simulink model "VTS_challenge_2021"  (R2019b)
settings: Solver=ode1  StartTime=0.0  StopTime=SIMULPARAM.T_end  FixedStep=SIMULPARAM.Ts  RelTol=1e-3
undefined symbols (not defined in the file or in its folder): BAT, CHAp, EM1, EM2, EMS, MTp, RDp, Speed_control, SPEEDCONTROL
libraries: simulink x3
(part 1 of 2)
settings Model: Creator=baohu  LastModifiedBy=HIEU
settings DataIOCC: ReturnWorkspaceOutputs=off
settings OptimizationCC: LifeSpan=inf
settings DebuggingCC: SFExecutionAtInitializationDiag=none  ArithmeticOperatorsInVariantConditions=warning
settings HardwareCC: ProdBitPerSizeT=32  ProdBitPerPtrDiffT=32  ProdWordSize=32  ProdHWDeviceType=Specified
settings ModelReferenceCC: EnableRefExpFcnMdlSchedulingChecks=off
settings SFSimCC: SimUseLocalCustomCode=off  CustomCodeUndefinedFunction=UseInterfaceOnly
settings RTWCC: RTWUseLocalCustomCode=off
settings CodeAppCC: StateflowObjectComments=on

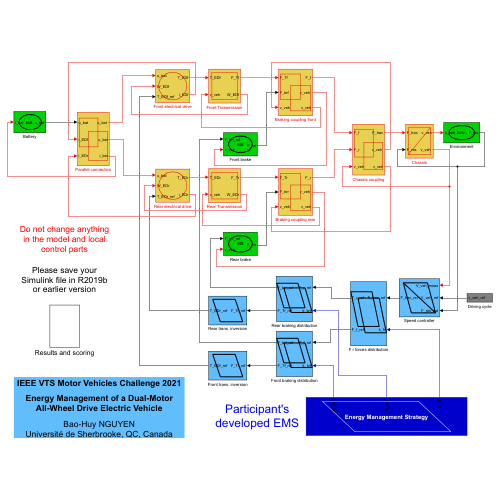
[thumbnail: Simulink's stored preview of the top-level diagram]
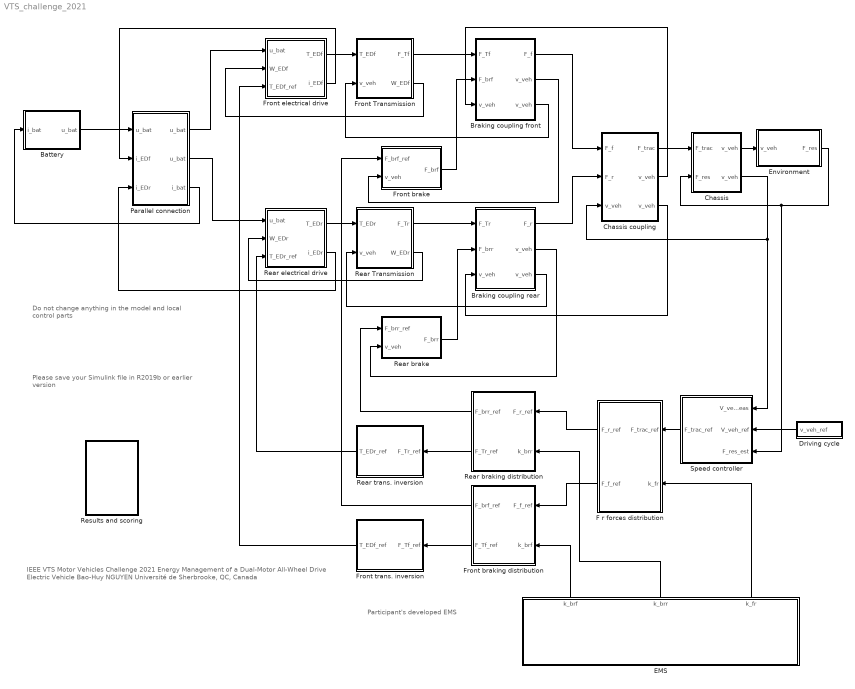
== system VTS_challenge_2021 ==
  note: Do not change anything in the model and local control parts
  note: Participant's developed EMS
  note: IEEE VTS Motor Vehicles Challenge 2021
      |
      | Energy Management of a Dual-Motor
      | All-Wheel Drive Electric Vehicle
      |
      | Bao-Huy NGUYEN
      | Université de Sherbrooke, QC, Canada
  note: Please save your Simulink file in R2019b or earlier version
  Battery : Subsystem
      mask Display:
      | plot(0,0,100,100, 1.2*[50,57.68,60.77,63.08,64.97,66.58,68,69.26,70.4, 	71.42,72.36,78.28,80,78.28,72.36,71.42,70.4, 	69.26,68,66.58,64.97,63.08,60.77,57.68,50,42.32, 	39.23,36.92,35.03,33.42,32,30.74,29.6,28.58, 	27.64,21.72,20,21.72,27.64,28.58,29.6,30.74,32, 	33.42,35.03,36.92,39.23,42.32,50]-10, 1.2*[20,21,22,23,24,25,26,27,28,29,30,40,50,60,70,71,72, 	73,74,75,76,77,78,79,80,79,78,77,76,75,74,73,72, 	71,70,60,50,40,30,29,28,27,26,25,24,23,22,21,20]-10)
      | disp('Bat.')
  Braking coupling front : Subsystem  mask(CM){}
      mask Display: plot(0,0,100,100,[35,35,95,95,35],[65,10,10,65,65], [5,5,65,65,5],[90,35,35,90,90])
  Braking coupling rear : Subsystem  mask(CM){}
      mask Display: plot(0,0,100,100,[35,35,95,95,35],[65,10,10,65,65], [5,5,65,65,5],[90,35,35,90,90])
  Chassis : Subsystem  mask(CM){}
      mask Display: plot(0,0,100,100,[10,10,90,90,10],[90,10,10,90,90], [10,90],[10,90])
  Chassis coupling : Subsystem  mask(CM){}
      mask Display: plot(0,0,100,100,[35,35,95,95,35],[65,10,10,65,65], [5,5,65,65,5],[90,35,35,90,90])
  Driving cycle : Subsystem
  EMS : Subsystem
      mask Display:
      | color('white');
      | plot(0,0,100,100,[10,30,90,70,10],[90,10,10,90,90])
      | disp('Energy Management Strategy')
  Environment : Subsystem
      mask Display:
      | plot(0,0,100,100, 1.2*[50,57.68,60.77,63.08,64.97,66.58,68,69.26,70.4, 	71.42,72.36,78.28,80,78.28,72.36,71.42,70.4, 	69.26,68,66.58,64.97,63.08,60.77,57.68,50,42.32, 	39.23,36.92,35.03,33.42,32,30.74,29.6,28.58, 	27.64,21.72,20,21.72,27.64,28.58,29.6,30.74,32, 	33.42,35.03,36.92,39.23,42.32,50]-10, 1.2*[20,21,22,23,24,25,26,27,28,29,30,40,50,60,70,71,72, 	73,74,75,76,77,78,79,80,79,78,77,76,75,74,73,72, 	71,70,60,50,40,30,29,28,27,26,25,24,23,22,21,20]-10)
      | disp('Env.')
  F r forces distribution : Subsystem
      mask Display: plot(0,0,100,100,[20,40,100,80,20],[75,20,20,75,75], [0,20,80,60,0],[85,30,30,85,85])
  Front Transmission : Subsystem
      mask Display: plot(0,0,100,100,[10,10,90,90,10],[90,10,10,90,90])
  Front brake : Subsystem
      mask Display:
      | plot(0,0,100,100, 1.2*[50,57.68,60.77,63.08,64.97,66.58,68,69.26,70.4, 	71.42,72.36,78.28,80,78.28,72.36,71.42,70.4, 	69.26,68,66.58,64.97,63.08,60.77,57.68,50,42.32, 	39.23,36.92,35.03,33.42,32,30.74,29.6,28.58, 	27.64,21.72,20,21.72,27.64,28.58,29.6,30.74,32, 	33.42,35.03,36.92,39.23,42.32,50]-10, 1.2*[20,21,22,23,24,25,26,27,28,29,30,40,50,60,70,71,72, 	73,74,75,76,77,78,79,80,79,78,77,76,75,74,73,72, 	71,70,60,50,40,30,29,28,27,26,25,24,23,22,21,20]-10)
      | disp('MS')
  Front braking distribution : Subsystem
      mask Display: plot(0,0,100,100,[20,40,100,80,20],[75,20,20,75,75], [0,20,80,60,0],[85,30,30,85,85])
  Front electrical drive : Subsystem
      mask Display: plot(0,0,100,100, 1.4*[50,57.68,60.77,63.08,64.97,66.58,68,69.26,70.4, 	71.42,72.36,78.28,80,78.28,72.36,71.42,70.4, 	69.26,68,66.58,64.97,63.08,60.77,57.68,50,42.32, 	39.23,36.92,35.03,33.42,32,30.74,29.6,28.58, 	27.64,21.72,20,21.72,27.64,28.58,29.6,30.74,32, 	33.42,35.03,36.92,39.23,42.32,50]-20, 1.4*[20,21,22,23,24,25,26,27,28,29,30,40,50,60,70,71,72, 	73,74,75,76,77,78,79,80,79,78,77,76,75,74,73,72, 	71,70,60,50,40,30,29,28,27,26,25,24,23,22,21,20]-20)
  Front trans. inversion : Subsystem
      mask Display: plot(0,0,100,100,[10,30,90,70,10],[90,10,10,90,90])
  Parallel connection : Subsystem  mask(CM){}
      mask Display: plot(0,0,100,100,[35,35,95,95,35],[65,10,10,65,65], [5,5,65,65,5],[90,35,35,90,90])
  Rear Transmission : Subsystem
      mask Display: plot(0,0,100,100,[10,10,90,90,10],[90,10,10,90,90])
  Rear brake : Subsystem
      mask Display:
      | plot(0,0,100,100, 1.2*[50,57.68,60.77,63.08,64.97,66.58,68,69.26,70.4, 	71.42,72.36,78.28,80,78.28,72.36,71.42,70.4, 	69.26,68,66.58,64.97,63.08,60.77,57.68,50,42.32, 	39.23,36.92,35.03,33.42,32,30.74,29.6,28.58, 	27.64,21.72,20,21.72,27.64,28.58,29.6,30.74,32, 	33.42,35.03,36.92,39.23,42.32,50]-10, 1.2*[20,21,22,23,24,25,26,27,28,29,30,40,50,60,70,71,72, 	73,74,75,76,77,78,79,80,79,78,77,76,75,74,73,72, 	71,70,60,50,40,30,29,28,27,26,25,24,23,22,21,20]-10)
      | disp('MS')
  Rear braking distribution : Subsystem
      mask Display: plot(0,0,100,100,[20,40,100,80,20],[75,20,20,75,75], [0,20,80,60,0],[85,30,30,85,85])
  Rear electrical drive : Subsystem
      mask Display: plot(0,0,100,100, 1.4*[50,57.68,60.77,63.08,64.97,66.58,68,69.26,70.4, 	71.42,72.36,78.28,80,78.28,72.36,71.42,70.4, 	69.26,68,66.58,64.97,63.08,60.77,57.68,50,42.32, 	39.23,36.92,35.03,33.42,32,30.74,29.6,28.58, 	27.64,21.72,20,21.72,27.64,28.58,29.6,30.74,32, 	33.42,35.03,36.92,39.23,42.32,50]-20, 1.4*[20,21,22,23,24,25,26,27,28,29,30,40,50,60,70,71,72, 	73,74,75,76,77,78,79,80,79,78,77,76,75,74,73,72, 	71,70,60,50,40,30,29,28,27,26,25,24,23,22,21,20]-20)
  Rear trans. inversion : Subsystem
      mask Display: plot(0,0,100,100,[10,30,90,70,10],[90,10,10,90,90])
  Results and scoring : Subsystem
  Speed controller : Subsystem
      mask Display: plot(0,0,100,100, [10,30,90,70,10,90],[90,10,10,90,90,10])
  wires:
  Environment/1(F_res) -> Chassis/2(F_res), Speed controller/3(F_res_est)
  Chassis/1(v_veh) -> Environment/1(v_veh)
  Speed controller/1(F_trac_ref) -> F r forces distribution/1(F_trac_ref)
  Chassis/2("v_veh ") -> Chassis coupling/3(v_veh), Speed controller/1(V_veh_meas)
  Front Transmission/2(W_EDf) -> Front electrical drive/2(W_EDf)
  Battery/1(u_bat) -> Parallel connection/1(u_bat)
  Parallel connection/3(i_bat) -> Battery/1(i_bat)
  Rear electrical drive/2(i_EDr) -> Parallel connection/3(i_EDr)
  Front electrical drive/2(i_EDf) -> Parallel connection/2("i_EDf  ")
  Parallel connection/1("u_bat ") -> Front electrical drive/1(u_bat)
  Parallel connection/2(" u_bat") -> Rear electrical drive/1(u_bat)
  Front electrical drive/1(T_EDf) -> Front Transmission/1(T_EDf)
  Rear electrical drive/1(T_EDr) -> Rear Transmission/1(T_EDr)
  Rear Transmission/2(W_EDr) -> Rear electrical drive/2(W_EDr)
  Front Transmission/1(F_Tf) -> Braking coupling front/1(F_Tf)
  Front brake/1(F_brf) -> Braking coupling front/2(F_brf)
  Braking coupling front/3(" v_veh") -> Front Transmission/2(v_veh)
  Rear Transmission/1(F_Tr) -> Braking coupling rear/1(F_Tr)
  Rear brake/1(F_brr) -> Braking coupling rear/2(F_brr)
  Braking coupling rear/3(" v_veh") -> Rear Transmission/2(v_veh)
  Braking coupling rear/2("v_veh ") -> Rear brake/2(v_veh)
  Braking coupling front/2("v_veh ") -> Front brake/2(v_veh)
  Braking coupling front/1(F_f) -> Chassis coupling/1(F_f)
  Braking coupling rear/1(F_r) -> Chassis coupling/2(F_r)
  Chassis coupling/1(F_trac) -> Chassis/1(F_trac)
  Chassis coupling/2("v_veh ") -> Braking coupling front/3(v_veh)
  Chassis coupling/3(" v_veh") -> Braking coupling rear/3(v_veh)
  Front braking distribution/2(F_Tf_ref) -> Front trans. inversion/1(F_Tf_ref)
  Rear braking distribution/2(F_Tr_ref) -> Rear trans. inversion/1(F_Tr_ref)
  Rear trans. inversion/1(T_EDr_ref) -> Rear electrical drive/3(T_EDr_ref)
  Front trans. inversion/1(T_EDf_ref) -> Front electrical drive/3(T_EDf_ref)
  F r forces distribution/1(F_r_ref) -> Rear braking distribution/1(F_r_ref)
  F r forces distribution/2(F_f_ref) -> Front braking distribution/1(F_f_ref)
  Rear braking distribution/1(F_brr_ref) -> Rear brake/1(F_brr_ref)
  Front braking distribution/1(F_brf_ref) -> Front brake/1(F_brf_ref)
  EMS/3(k_fr) -> F r forces distribution/2(k_fr)
  EMS/2(k_brr) -> Rear braking distribution/2(k_brr)
  EMS/1(k_brf) -> Front braking distribution/2(k_brf)
  Driving cycle/1(v_veh_ref) -> Speed controller/2(V_veh_ref)

== system VTS_challenge_2021/Battery ==
  i_bat : Inport
  Air : Subsystem
      mask Display: plot(0,0,100,100, 1.2*[50,57.68,60.77,63.08,64.97,66.58,68,69.26,70.4, 	71.42,72.36,78.28,80,78.28,72.36,71.42,70.4, 	69.26,68,66.58,64.97,63.08,60.77,57.68,50,42.32, 	39.23,36.92,35.03,33.42,32,30.74,29.6,28.58, 	27.64,21.72,20,21.72,27.64,28.58,29.6,30.74,32, 	33.42,35.03,36.92,39.23,42.32,50]-10, 1.2*[20,21,22,23,24,25,26,27,28,29,30,40,50,60,70,71,72, 	73,74,75,76,77,78,79,80,79,78,77,76,75,74,73,72, 	71,70,60,50,40,30,29,28,27,26,25,24,23,22,21,20]-10)
  Cell ESR : Subsystem  mask(CM){}
      mask Display: plot(0,0,100,100, [50,57.68,60.77,63.08,64.97,66.58,68,69.26,70.4, 	71.42,72.36,78.28,80,78.28,72.36,71.42,70.4, 	69.26,68,66.58,64.97,63.08,60.77,57.68,50,42.32, 	39.23,36.92,35.03,33.42,32,30.74,29.6,28.58, 	27.64,21.72,20,21.72,27.64,28.58,29.6,30.74,32, 	33.42,35.03,36.92,39.23,42.32,50], [20,21,22,23,24,25,26,27,28,29,30,40,50,60,70,71,72, 	73,74,75,76,77,78,79,80,79,78,77,76,75,74,73,72, 	71,70,60,50,40,30,29,28,27,26,25,24,23,22,21,20]-15,  [50,57.68,60.77,63.08,64.97,66.58,68,69.26,70.4, 	71.42,72.36,78.28,80,78.28,72.36,71.42,70.4, 	69.26,68,66.58,64.97,63.08,60.77,57.68,50,42.32, 	39.23,36.92,35.03,33.42,32,30.74,29.6,28.58, 	27.64,21.72,20,21.72,27.64,28.58,29.6,30.74,32, 	33.42,35.03,36.92,39.23,42.32,50], [20,21,22,23,24,25,26,27,28,29,30,40,50,60,70,71,72, 	73,74,75,76,77,78,79,80,79,78,77,76,75,74,73,72, 	71,70,60,50,40,30,29,28,27,26,25,24,23,22,21,20]+15)
  Cell OCV : Subsystem
      mask Display: plot(0,0,100,100, 1.2*[50,57.68,60.77,63.08,64.97,66.58,68,69.26,70.4, 	71.42,72.36,78.28,80,78.28,72.36,71.42,70.4, 	69.26,68,66.58,64.97,63.08,60.77,57.68,50,42.32, 	39.23,36.92,35.03,33.42,32,30.74,29.6,28.58, 	27.64,21.72,20,21.72,27.64,28.58,29.6,30.74,32, 	33.42,35.03,36.92,39.23,42.32,50]-10, 1.2*[20,21,22,23,24,25,26,27,28,29,30,40,50,60,70,71,72, 	73,74,75,76,77,78,79,80,79,78,77,76,75,74,73,72, 	71,70,60,50,40,30,29,28,27,26,25,24,23,22,21,20]-10)
  Series parallel connection : Subsystem  mask(CM){}
      mask Display: plot(0,0,100,100, [10,10,90,90,10],[90,10,10,90,90], [10,90,10],[10,45,90])
  Thermal capacitance : Subsystem  mask(CM){}
      mask Display: plot(0,0,100,100,[10,10,90,90,10],[90,10,10,90,90], [10,90],[10,90])
  Thermal resistance : Subsystem
      mask Display: plot(0,0,100,100,[10,10,90,90,10],[90,10,10,90,90])
  u_bat : Outport  InitialOutput=0
  tag scope: i_bat=global, u_bat=global
  wires:
  i_bat/1 -> Series parallel connection/2(i_bat), [i_bat]
  Series parallel connection/1(u_bat) -> u_bat/1, [u_bat]
  Cell ESR/1(u_cell) -> Series parallel connection/1(u_cell)
  Series parallel connection/2("i_cell ") -> Cell ESR/3("i_cell ")
  Cell OCV/1(u_cell_OC) -> Cell ESR/1(u_cell_OC)
  Cell ESR/3(i_cell) -> Cell OCV/1(i_cell)
  Thermal resistance/1(q_sa) -> Air/1(q_sa)
  Air/1(T_air) -> Thermal resistance/2(T_air)
  Thermal resistance/2(q_cs) -> Thermal capacitance/2(q_cs)
  Thermal capacitance/1(T_cell) -> Thermal resistance/1(T_cell)
  Thermal capacitance/2(" T_cell ") -> Cell ESR/2(T_cell)
  Cell ESR/2(q_cell) -> Thermal capacitance/1(q_cell)

== system VTS_challenge_2021/Braking coupling front ==
  F_Tf : Inport
  F_brf : Inport  Port=2
  v_veh : Inport  Port=3
  Sum : Sum  Inputs=|++
  F_f : Outport  InitialOutput=0
  "v_veh " : Outport  Port=2  InitialOutput=0
  " v_veh" : Outport  Port=3  InitialOutput=0
  tag scope: F_Tf=global, F_brf=global, F_f=global
  wires:
  v_veh/1 -> " v_veh"/1, "v_veh "/1
  Sum/1 -> [F_f], F_f/1
  F_brf/1 -> [F_brf], Sum/2
  F_Tf/1 -> [F_Tf], Sum/1

== system VTS_challenge_2021/Braking coupling rear ==
  F_Tr : Inport
  F_brr : Inport  Port=2
  v_veh : Inport  Port=3
  Sum : Sum  Inputs=|++
  F_r : Outport  InitialOutput=0
  "v_veh " : Outport  Port=2  InitialOutput=0
  " v_veh" : Outport  Port=3  InitialOutput=0
  tag scope: F_Tr=global, F_brr=global, F_r=global
  wires:
  F_Tr/1 -> [F_Tr], Sum/1
  F_brr/1 -> [F_brr], Sum/2
  Sum/1 -> [F_r], F_r/1
  v_veh/1 -> "v_veh "/1, " v_veh"/1

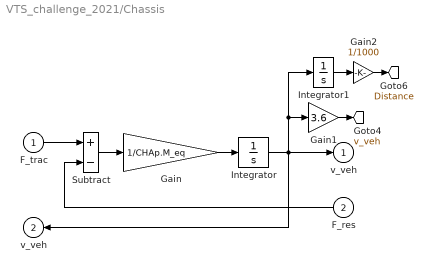
== system VTS_challenge_2021/Chassis ==
  F_trac : Inport
  F_res : Inport  Port=2
  Gain : Gain  Gain=1/CHAp.M_eq
  Gain1 : Gain  Gain=3.6
  Gain2 : Gain  Gain=1/1000
  Integrator : Integrator
  Integrator1 : Integrator
  Subtract : Sum  Inputs=+-
  v_veh : Outport  InitialOutput=0
  "v_veh " : Outport  Port=2  InitialOutput=0
  tag scope: Distance=global, v_veh=global
  wires:
  F_trac/1 -> Subtract/1
  F_res/1 -> Subtract/2
  Subtract/1 -> Gain/1
  Gain/1 -> Integrator/1
  Gain1/1 -> [v_veh]
  Integrator1/1 -> Gain2/1
  Integrator/1 -> v_veh/1, Gain1/1, Integrator1/1, "v_veh "/1
  Gain2/1 -> [Distance]

== system VTS_challenge_2021/Chassis coupling ==
  F_f : Inport
  F_r : Inport  Port=2
  v_veh : Inport  Port=3
  Sum : Sum  Inputs=|++
  F_trac : Outport  InitialOutput=0
  "v_veh " : Outport  Port=2  InitialOutput=0
  " v_veh" : Outport  Port=3  InitialOutput=0
  tag scope: F_trac=global
  wires:
  v_veh/1 -> " v_veh"/1, "v_veh "/1
  F_r/1 -> Sum/2
  F_f/1 -> Sum/1
  Sum/1 -> [F_trac], F_trac/1

== system VTS_challenge_2021/Driving cycle ==
  Driving cycle : simulink/Sources/Repeating Sequence  rep_seq_t=CYCL.time  rep_seq_y=CYCL.velocity  mask(Repeating table){}
  Gain1 : Gain  Gain=1/3.6
  Saturation : Saturate  UpperLimit=100  LowerLimit=0
  v_veh_ref : Outport
  wires:
  Gain1/1 -> v_veh_ref/1
  Driving cycle/1 -> Saturation/1
  Saturation/1 -> Gain1/1

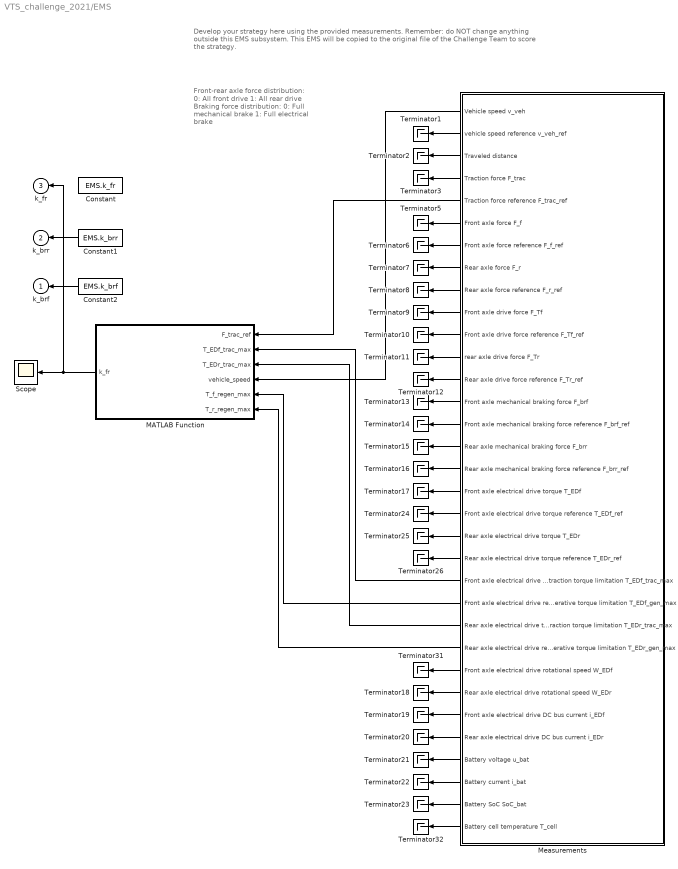
== system VTS_challenge_2021/EMS ==
  note: Front-rear axle force distribution:
      | 0: All front drive
      | 1: All rear drive
      |
      | Braking force distribution:
      | 0: Full mechanical brake
      | 1: Full electrical brake
  note: Develop your strategy here using the provided measurements.
      |
      | Remember: do NOT change anything outside this EMS subsystem. This EMS will be copied to the original file of the Challenge Team to score the strategy.
  Constant : Constant  Value=EMS.k_fr
  Constant1 : Constant  Value=EMS.k_brr
  Constant2 : Constant  Value=EMS.k_brf
  MATLAB Function : MATLAB Function  TreatAsAtomicUnit=on  SystemSampleTime=0.01
  Measurements : Subsystem
  Scope : Scope
  Terminator{1..3,5..26,31..32} (27 alike) : Terminator
  k_brf : Outport  InitialOutput=0
  k_brr : Outport  Port=2  InitialOutput=0
  k_fr : Outport  Port=3  InitialOutput=0
  wires:
  Constant1/1 -> k_brr/1
  Constant2/1 -> k_brf/1
  Measurements/2(vehicle speed reference v_veh_ref) -> Terminator1/1
  Measurements/3(Traveled distance) -> Terminator2/1
  Measurements/4(Traction force F_trac) -> Terminator3/1
  Measurements/6(Front axle force F_f) -> Terminator5/1
  Measurements/7(Front axle force reference F_f_ref) -> Terminator6/1
  Measurements/8(Rear axle force F_r) -> Terminator7/1
  Measurements/9(Rear axle force reference F_r_ref) -> Terminator8/1
  Measurements/10(Front axle drive force F_Tf) -> Terminator9/1
  Measurements/11(Front axle drive force reference F_Tf_ref) -> Terminator10/1
  Measurements/12(rear axle drive force F_Tr) -> Terminator11/1
  Measurements/13(Rear axle drive force reference F_Tr_ref) -> Terminator12/1
  Measurements/14(Front axle mechanical braking force F_brf) -> Terminator13/1
  Measurements/15(Front axle mechanical braking force reference F_brf_ref) -> Terminator14/1
  Measurements/16(Rear axle mechanical braking force F_brr) -> Terminator15/1
  Measurements/17(Rear axle mechanical braking force reference F_brr_ref) -> Terminator16/1
  Measurements/18(Front axle electrical drive torque T_EDf) -> Terminator17/1
  Measurements/19(Front axle electrical drive torque reference T_EDf_ref) -> Terminator24/1
  Measurements/20(Rear axle electrical drive torque T_EDr) -> Terminator25/1
  Measurements/21(Rear axle electrical drive torque reference T_EDr_ref) -> Terminator26/1
  Measurements/26(Front axle electrical drive rotational speed W_EDf) -> Terminator31/1
  Measurements/27(Rear axle electrical drive rotational speed W_EDr) -> Terminator18/1
  Measurements/28(Front axle electrical drive DC bus current i_EDf) -> Terminator19/1
  Measurements/29(Rear axle electrical drive DC bus current i_EDr) -> Terminator20/1
  Measurements/30(Battery voltage u_bat) -> Terminator21/1
  Measurements/31(Battery current i_bat) -> Terminator22/1
  Measurements/32(Battery SoC SoC_bat) -> Terminator23/1
  Measurements/33(Battery cell temperature T_cell) -> Terminator32/1
  Measurements/1(Vehicle speed v_veh) -> MATLAB Function/4(vehicle_speed)
  MATLAB Function/1(k_fr) -> Scope/1, k_fr/1
  Measurements/5(Traction force reference F_trac_ref) -> MATLAB Function/1(F_trac_ref)
  Measurements/22(Front axle electrical drive traction torque limitation T_EDf_trac_max) -> MATLAB Function/2(T_EDf_trac_max)
  Measurements/24(Rear axle electrical drive traction torque limitation T_EDr_trac_max) -> MATLAB Function/3(T_EDr_trac_max)
  Measurements/23(Front axle electrical drive regenerative torque limitation T_EDf_gen_max) -> MATLAB Function/5(T_f_regen_max)
  Measurements/25(Rear axle electrical drive regenerative torque limitation T_EDr_gen_max) -> MATLAB Function/6(T_r_regen_max)

== system VTS_challenge_2021/Environment ==
  v_veh : Inport
  Abs : Abs
  Add : Sum
  Fcn : Fcn  Expr=RDp.Kaero*(u+0)^2
  Product : Product  RndMeth=Zero
  Saturation : Saturate  UpperLimit=1  LowerLimit=0
  pente de 10%1 : Constant  Value=RDp.F_sec
  F_res : Outport  InitialOutput=0
  wires:
  v_veh/1 -> Fcn/1, Abs/1
  Add/1 -> F_res/1
  Fcn/1 -> Add/1
  pente de 10%1/1 -> Product/2
  Product/1 -> Add/2
  Abs/1 -> Saturation/1
  Saturation/1 -> Product/1

== system VTS_challenge_2021/F r forces distribution ==
  F_trac_ref : Inport
  k_fr : Inport  Port=2
  Constant : Constant
  Product : Product  RndMeth=Zero
  Product1 : Product  RndMeth=Zero
  Sum : Sum  Inputs=+-
  F_r_ref : Outport  InitialOutput=0
  F_f_ref : Outport  Port=2  InitialOutput=0
  tag scope: F_f_ref=global, F_r_ref=global
  wires:
  Constant/1 -> Sum/1
  k_fr/1 -> Sum/2, Product1/2
  F_trac_ref/1 -> Product/1, Product1/1
  Sum/1 -> Product/2
  Product/1 -> [F_r_ref], F_r_ref/1
  Product1/1 -> [F_f_ref], F_f_ref/1

== system VTS_challenge_2021/Front Transmission ==
  T_EDf : Inport
  v_veh : Inport  Port=2
  Gain : Gain  Gain=MTp.k_tran_f
  Gain1 : Gain  Gain=MTp.k_tran_f
  Product2 : Product  RndMeth=Zero
  Regenerative : Gain  Gain=1/MTp.Gear_eff
  Switch : Switch
  Traction : Gain  Gain=MTp.Gear_eff
  F_Tf : Outport  InitialOutput=0
  W_EDf : Outport  Port=2  InitialOutput=0
  wires:
  Switch/1 -> Gain/1
  Regenerative/1 -> Switch/3
  Traction/1 -> Switch/1
  Product2/1 -> Switch/2
  v_veh/1 -> Gain1/1
  Gain1/1 -> Product2/2, W_EDf/1
  Gain/1 -> F_Tf/1
  T_EDf/1 -> Traction/1, Regenerative/1, Product2/1

== system VTS_challenge_2021/Front brake ==
  F_brf_ref : Inport
  v_veh : Inport  Port=2
  Saturation : Saturate  UpperLimit=0  LowerLimit=-inf
  Terminator : Terminator
  F_brf : Outport  InitialOutput=0
  wires:
  Saturation/1 -> F_brf/1
  v_veh/1 -> Terminator/1
  F_brf_ref/1 -> Saturation/1

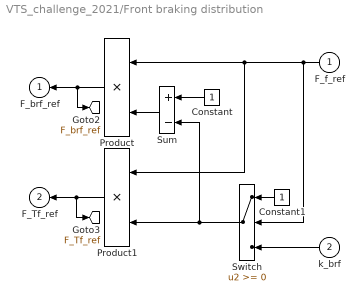
== system VTS_challenge_2021/Front braking distribution ==
  F_f_ref : Inport
  k_brf : Inport  Port=2
  Constant : Constant
  Constant1 : Constant
  Product : Product  RndMeth=Zero
  Product1 : Product  RndMeth=Zero
  Sum : Sum  Inputs=+-
  Switch : Switch
  F_brf_ref : Outport  InitialOutput=0
  F_Tf_ref : Outport  Port=2  InitialOutput=0
  tag scope: F_Tf_ref=global, F_brf_ref=global
  wires:
  Constant/1 -> Sum/1
  Switch/1 -> Sum/2, Product1/2
  F_f_ref/1 -> Switch/2, Product/1, Product1/1
  Sum/1 -> Product/2
  Product/1 -> [F_brf_ref], F_brf_ref/1
  Product1/1 -> [F_Tf_ref], F_Tf_ref/1
  Constant1/1 -> Switch/1
  k_brf/1 -> Switch/3

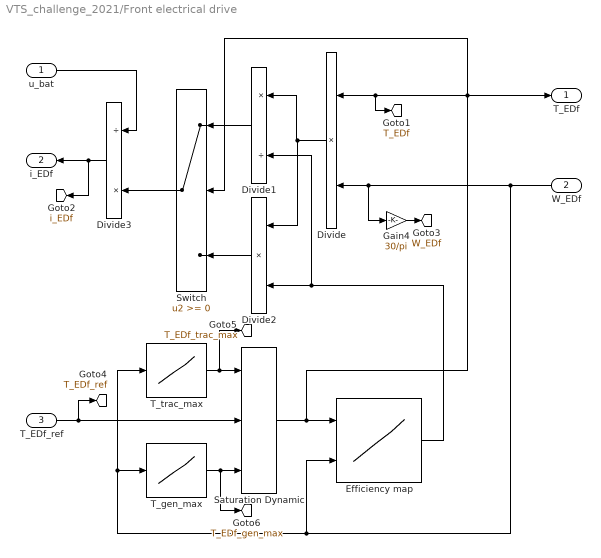
== system VTS_challenge_2021/Front electrical drive ==
  u_bat : Inport
  W_EDf : Inport  Port=2
  T_EDf_ref : Inport  Port=3
  Divide : Product  Inputs=**
  Divide1 : Product  Inputs=*/
  Divide2 : Product  Inputs=**
  Divide3 : Product  Inputs=/*
  Efficiency map : Lookup_n-D  BreakpointsForDimension1=EM1.Torque  BreakpointsForDimension2=EM1.Speed  Table=EM1.Eff  InterpMethod=Cubic spline  ExtrapMethod=Cubic spline  InternalRulePriority=Speed  RndMeth=Simplest  InputSameDT=on
  Gain4 : Gain  Gain=30/pi
  Saturation Dynamic : simulink/Discontinuities/Saturation Dynamic  OutMin=[]  OutMax=[]  OutDataTypeStr=Inherit: Same as second input  OutDataType=fixdt(1, 16)  OutScaling=2^-10  DoSatur=off
  Switch : Switch
  T_gen_max : Lookup_n-D  NumberOfTableDimensions=1  BreakpointsForDimension1=EM1.Speed  Table=EM1.T_gen_max  InternalRulePriority=Speed  RndMeth=Simplest  InputSameDT=on
  T_trac_max : Lookup_n-D  NumberOfTableDimensions=1  BreakpointsForDimension1=EM1.Speed  Table=EM1.T_trac_max  InternalRulePriority=Speed  RndMeth=Simplest  InputSameDT=on
  T_EDf : Outport
  i_EDf : Outport  Port=2
  tag scope: T_EDf=global, T_EDf_gen_max=global, T_EDf_ref=global, T_EDf_trac_max=global, W_EDf=global, i_EDf=global
  wires:
  Divide3/1 -> [i_EDf], i_EDf/1
  Divide/1 -> Divide1/1, Divide2/1
  Divide1/1 -> Switch/1
  T_EDf_ref/1 -> [T_EDf_ref], Saturation Dynamic/2
  Divide2/1 -> Switch/3
  Efficiency map/1 -> Divide1/2, Divide2/2
  u_bat/1 -> Divide3/1
  Switch/1 -> Divide3/2
  Gain4/1 -> [W_EDf]
  W_EDf/1 -> Efficiency map/2, T_gen_max/1, T_trac_max/1, Gain4/1, Divide/2
  Saturation Dynamic/1 -> Switch/2, T_EDf/1, [T_EDf], Divide/1, Efficiency map/1
  T_trac_max/1 -> [T_EDf_trac_max], Saturation Dynamic/1
  T_gen_max/1 -> [T_EDf_gen_max], Saturation Dynamic/3

== system VTS_challenge_2021/Front trans. inversion ==
  F_Tf_ref : Inport
  K_cm : Gain  Gain=1/MTp.k_tran_f  SaturateOnIntegerOverflow=on  OutDataTypeStr=Inherit: Same as input  ParamDataTypeStr=Inherit: Same as input
  T_EDf_ref : Outport  InitialOutput=0
  wires:
  F_Tf_ref/1 -> K_cm/1
  K_cm/1 -> T_EDf_ref/1

== system VTS_challenge_2021/Parallel connection ==
  u_bat : Inport
  "i_EDf  " : Inport  Port=2
  i_EDr : Inport  Port=3
  Sum : Sum  Inputs=|++
  "u_bat " : Outport  InitialOutput=0
  " u_bat" : Outport  Port=2  InitialOutput=0
  i_bat : Outport  Port=3  InitialOutput=0
  wires:
  u_bat/1 -> " u_bat"/1, "u_bat "/1
  "i_EDf  "/1 -> Sum/1
  i_EDr/1 -> Sum/2
  Sum/1 -> i_bat/1

== system VTS_challenge_2021/Rear Transmission ==
  T_EDr : Inport
  v_veh : Inport  Port=2
  Gain : Gain  Gain=MTp.k_tran_r
  Gain1 : Gain  Gain=MTp.k_tran_r
  Product2 : Product  RndMeth=Zero
  Regenerative : Gain  Gain=1/MTp.Gear_eff
  Switch : Switch
  Traction : Gain  Gain=MTp.Gear_eff
  F_Tr : Outport  InitialOutput=0
  W_EDr : Outport  Port=2  InitialOutput=0
  wires:
  T_EDr/1 -> Product2/1, Regenerative/1, Traction/1
  Gain/1 -> F_Tr/1
  Gain1/1 -> W_EDr/1, Product2/2
  v_veh/1 -> Gain1/1
  Product2/1 -> Switch/2
  Traction/1 -> Switch/1
  Regenerative/1 -> Switch/3
  Switch/1 -> Gain/1

== system VTS_challenge_2021/Rear brake ==
  F_brr_ref : Inport
  v_veh : Inport  Port=2
  Saturation : Saturate  UpperLimit=0  LowerLimit=-inf
  Terminator : Terminator
  F_brr : Outport  InitialOutput=0
  wires:
  F_brr_ref/1 -> Saturation/1
  v_veh/1 -> Terminator/1
  Saturation/1 -> F_brr/1

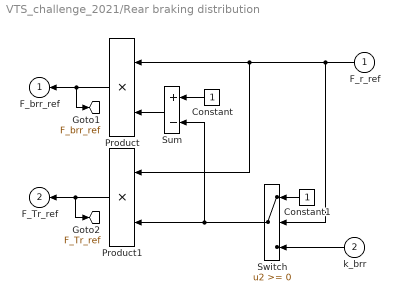
== system VTS_challenge_2021/Rear braking distribution ==
  F_r_ref : Inport
  k_brr : Inport  Port=2
  Constant : Constant
  Constant1 : Constant
  Product : Product  RndMeth=Zero
  Product1 : Product  RndMeth=Zero
  Sum : Sum  Inputs=+-
  Switch : Switch
  F_brr_ref : Outport  InitialOutput=0
  F_Tr_ref : Outport  Port=2  InitialOutput=0
  tag scope: F_Tr_ref=global, F_brr_ref=global
  wires:
  Product1/1 -> [F_Tr_ref], F_Tr_ref/1
  Product/1 -> [F_brr_ref], F_brr_ref/1
  Sum/1 -> Product/2
  F_r_ref/1 -> Switch/2, Product1/1, Product/1
  Switch/1 -> Product1/2, Sum/2
  Constant/1 -> Sum/1
  k_brr/1 -> Switch/3
  Constant1/1 -> Switch/1

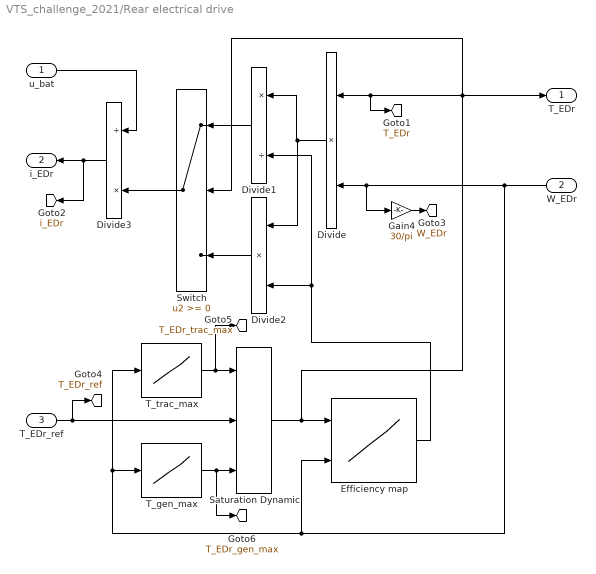
== system VTS_challenge_2021/Rear electrical drive ==
  u_bat : Inport
  W_EDr : Inport  Port=2
  T_EDr_ref : Inport  Port=3
  Divide : Product  Inputs=**
  Divide1 : Product  Inputs=*/
  Divide2 : Product  Inputs=**
  Divide3 : Product  Inputs=/*
  Efficiency map : Lookup_n-D  BreakpointsForDimension1=EM2.Torque  BreakpointsForDimension2=EM2.Speed  Table=EM2.Eff  InterpMethod=Cubic spline  ExtrapMethod=Cubic spline  InternalRulePriority=Speed  RndMeth=Simplest  InputSameDT=on
  Gain4 : Gain  Gain=30/pi
  Saturation Dynamic : simulink/Discontinuities/Saturation Dynamic  OutMin=[]  OutMax=[]  OutDataTypeStr=Inherit: Same as second input  OutDataType=fixdt(1, 16)  OutScaling=2^-10  DoSatur=off
  Switch : Switch
  T_gen_max : Lookup_n-D  NumberOfTableDimensions=1  BreakpointsForDimension1=EM2.Speed  Table=EM2.T_gen_max  InternalRulePriority=Speed  RndMeth=Simplest  InputSameDT=on
  T_trac_max : Lookup_n-D  NumberOfTableDimensions=1  BreakpointsForDimension1=EM2.Speed  Table=EM2.T_trac_max  InternalRulePriority=Speed  RndMeth=Simplest  InputSameDT=on
  T_EDr : Outport
  i_EDr : Outport  Port=2
  tag scope: T_EDr=global, T_EDr_gen_max=global, T_EDr_ref=global, T_EDr_trac_max=global, W_EDr=global, i_EDr=global
  wires:
  Switch/1 -> Divide3/2
  u_bat/1 -> Divide3/1
  Efficiency map/1 -> Divide2/2, Divide1/2
  Divide2/1 -> Switch/3
  Divide1/1 -> Switch/1
  Divide/1 -> Divide2/1, Divide1/1
  Divide3/1 -> [i_EDr], i_EDr/1
  Gain4/1 -> [W_EDr]
  T_gen_max/1 -> [T_EDr_gen_max], Saturation Dynamic/3
  Saturation Dynamic/1 -> T_EDr/1, Switch/2, [T_EDr], Divide/1, Efficiency map/1
  T_trac_max/1 -> [T_EDr_trac_max], Saturation Dynamic/1
  T_EDr_ref/1 -> [T_EDr_ref], Saturation Dynamic/2
  W_EDr/1 -> Efficiency map/2, T_gen_max/1, T_trac_max/1, Gain4/1, Divide/2

== system VTS_challenge_2021/Rear trans. inversion ==
  F_Tr_ref : Inport
  K_cm : Gain  Gain=1/MTp.k_tran_r  SaturateOnIntegerOverflow=on  OutDataTypeStr=Inherit: Same as input  ParamDataTypeStr=Inherit: Same as input
  T_EDr_ref : Outport  InitialOutput=0
  wires:
  K_cm/1 -> T_EDr_ref/1
  F_Tr_ref/1 -> K_cm/1

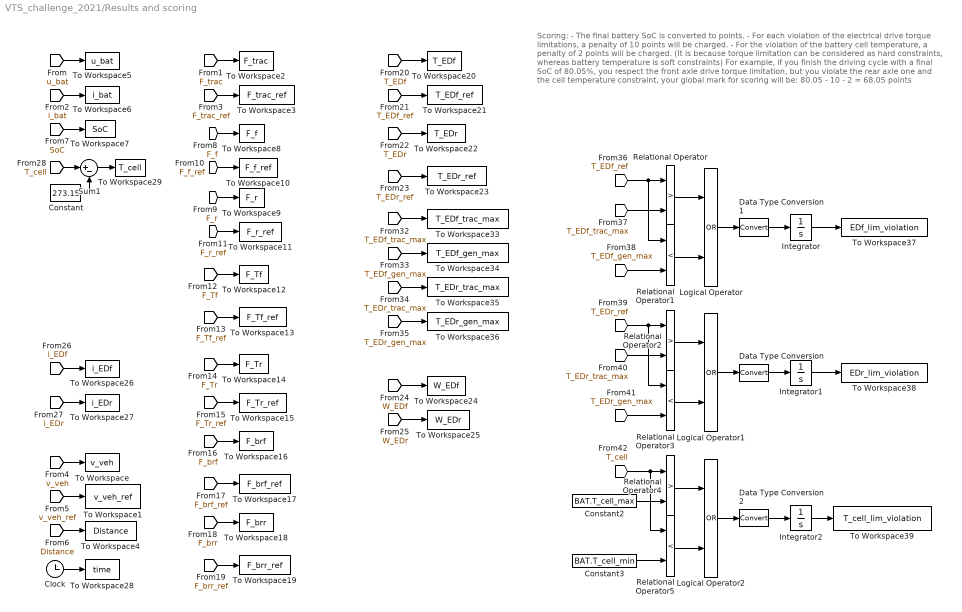
== system VTS_challenge_2021/Results and scoring ==
  note: Scoring:
      | - The final battery SoC is converted to points.
      | - For each violation of the electrical drive torque limitations, a penalty of 10 points will be charged.
      | - For the violation of the battery cell temperature, a penalty of 2 points will be charged.
      | (It is because torque limitation can be considered as hard constraints, whereas battery temperature is soft constraints)
      |
      | For example, if you finish the driving cycle with a final SoC of 80.05%, you respect the front axle drive torque limitation, but you violate the rear axle one and the cell temperature constraint, your global mark for scoring will be:
      | 80.05 - 10 - 2 = 68.05 points
  Clock : Clock
  Constant : Constant  Value=273.15
  Constant2 : Constant  Value=BAT.T_cell_max
  Constant3 : Constant  Value=BAT.T_cell_min
  Data Type Conversion : DataTypeConversion
  Data Type Conversion1 : DataTypeConversion
  Data Type Conversion2 : DataTypeConversion
  Integrator : Integrator
  Integrator1 : Integrator
  Integrator2 : Integrator
  Logical Operator : Logic  Operator=OR  AllPortsSameDT=off  OutDataTypeStr=boolean
  Logical Operator1 : Logic  Operator=OR  AllPortsSameDT=off  OutDataTypeStr=boolean
  Logical Operator2 : Logic  Operator=OR  AllPortsSameDT=off  OutDataTypeStr=boolean
  Relational Operator : RelationalOperator  Operator=>  OutDataTypeStr=boolean  RndMeth=Nearest
  Relational Operator1 : RelationalOperator  Operator=<  OutDataTypeStr=boolean  RndMeth=Nearest
  Relational Operator2 : RelationalOperator  Operator=>  OutDataTypeStr=boolean  RndMeth=Nearest
  Relational Operator3 : RelationalOperator  Operator=<  OutDataTypeStr=boolean  RndMeth=Nearest
  Relational Operator4 : RelationalOperator  Operator=>  OutDataTypeStr=boolean  RndMeth=Nearest
  Relational Operator5 : RelationalOperator  Operator=<  OutDataTypeStr=boolean  RndMeth=Nearest
  Sum1 : Sum  Inputs=|+-
  To Workspace : ToWorkspace  VariableName=v_veh  SampleTime=-1
      settings: Decimation=SIMULPARAM.Decimation
  To Workspace1 : ToWorkspace  VariableName=v_veh_ref  SampleTime=-1
      settings: Decimation=SIMULPARAM.Decimation
  To Workspace10 : ToWorkspace  VariableName=F_f_ref  SampleTime=-1
      settings: Decimation=SIMULPARAM.Decimation
  To Workspace11 : ToWorkspace  VariableName=F_r_ref  SampleTime=-1
      settings: Decimation=SIMULPARAM.Decimation
  To Workspace12 : ToWorkspace  VariableName=F_Tf  SampleTime=-1
      settings: Decimation=SIMULPARAM.Decimation
  To Workspace13 : ToWorkspace  VariableName=F_Tf_ref  SampleTime=-1
      settings: Decimation=SIMULPARAM.Decimation
  To Workspace14 : ToWorkspace  VariableName=F_Tr  SampleTime=-1
      settings: Decimation=SIMULPARAM.Decimation
  To Workspace15 : ToWorkspace  VariableName=F_Tr_ref  SampleTime=-1
      settings: Decimation=SIMULPARAM.Decimation
  To Workspace16 : ToWorkspace  VariableName=F_brf  SampleTime=-1
      settings: Decimation=SIMULPARAM.Decimation
  To Workspace17 : ToWorkspace  VariableName=F_brf_ref  SampleTime=-1
      settings: Decimation=SIMULPARAM.Decimation
  To Workspace18 : ToWorkspace  VariableName=F_brr  SampleTime=-1
      settings: Decimation=SIMULPARAM.Decimation
  To Workspace19 : ToWorkspace  VariableName=F_brr_ref  SampleTime=-1
      settings: Decimation=SIMULPARAM.Decimation
  To Workspace2 : ToWorkspace  VariableName=F_trac  SampleTime=-1
      settings: Decimation=SIMULPARAM.Decimation
  To Workspace20 : ToWorkspace  VariableName=T_EDf  SampleTime=-1
      settings: Decimation=SIMULPARAM.Decimation
  To Workspace21 : ToWorkspace  VariableName=T_EDf_ref  SampleTime=-1
      settings: Decimation=SIMULPARAM.Decimation
  To Workspace22 : ToWorkspace  VariableName=T_EDr  SampleTime=-1
      settings: Decimation=SIMULPARAM.Decimation
  To Workspace23 : ToWorkspace  VariableName=T_EDr_ref  SampleTime=-1
      settings: Decimation=SIMULPARAM.Decimation
  To Workspace24 : ToWorkspace  VariableName=W_EDf  SampleTime=-1
      settings: Decimation=SIMULPARAM.Decimation
  To Workspace25 : ToWorkspace  VariableName=W_EDr  SampleTime=-1
      settings: Decimation=SIMULPARAM.Decimation
  To Workspace26 : ToWorkspace  VariableName=i_EDf  SampleTime=-1
      settings: Decimation=SIMULPARAM.Decimation
  To Workspace27 : ToWorkspace  VariableName=i_EDr  SampleTime=-1
      settings: Decimation=SIMULPARAM.Decimation
  To Workspace28 : ToWorkspace  VariableName=time  SampleTime=-1
      settings: Decimation=SIMULPARAM.Decimation
  To Workspace29 : ToWorkspace  VariableName=T_cell  SampleTime=-1
      settings: Decimation=SIMULPARAM.Decimation
  To Workspace3 : ToWorkspace  VariableName=F_trac_ref  SampleTime=-1
      settings: Decimation=SIMULPARAM.Decimation
  To Workspace33 : ToWorkspace  VariableName=T_EDf_trac_max  SampleTime=-1
      settings: Decimation=SIMULPARAM.Decimation
  To Workspace34 : ToWorkspace  VariableName=T_EDf_gen_max  SampleTime=-1
      settings: Decimation=SIMULPARAM.Decimation
  To Workspace35 : ToWorkspace  VariableName=T_EDr_trac_max  SampleTime=-1
      settings: Decimation=SIMULPARAM.Decimation
  To Workspace36 : ToWorkspace  VariableName=T_EDr_gen_max  SampleTime=-1
      settings: Decimation=SIMULPARAM.Decimation
  To Workspace37 : ToWorkspace  VariableName=EDf_lim_violation  SampleTime=-1
      settings: Decimation=SIMULPARAM.Decimation
  To Workspace38 : ToWorkspace  VariableName=EDr_lim_violation  SampleTime=-1
      settings: Decimation=SIMULPARAM.Decimation
  To Workspace39 : ToWorkspace  VariableName=T_cell_lim_violation  SampleTime=-1
      settings: Decimation=SIMULPARAM.Decimation
  To Workspace4 : ToWorkspace  VariableName=Distance  SampleTime=-1
      settings: Decimation=SIMULPARAM.Decimation
  To Workspace5 : ToWorkspace  VariableName=u_bat  SampleTime=-1
      settings: Decimation=SIMULPARAM.Decimation
  To Workspace6 : ToWorkspace  VariableName=i_bat  SampleTime=-1
      settings: Decimation=SIMULPARAM.Decimation
  To Workspace7 : ToWorkspace  VariableName=SoC  SampleTime=-1
      settings: Decimation=SIMULPARAM.Decimation
  To Workspace8 : ToWorkspace  VariableName=F_f  SampleTime=-1
      settings: Decimation=SIMULPARAM.Decimation
  To Workspace9 : ToWorkspace  VariableName=F_r  SampleTime=-1
      settings: Decimation=SIMULPARAM.Decimation
  wires:
  [i_bat] -> To Workspace6/1
  [v_veh_ref] -> To Workspace1/1
  [v_veh] -> To Workspace/1
  [u_bat] -> To Workspace5/1
  [Distance] -> To Workspace4/1
  [SoC] -> To Workspace7/1
  [F_trac] -> To Workspace2/1
  [F_trac_ref] -> To Workspace3/1
  [F_f] -> To Workspace8/1
  [F_r] -> To Workspace9/1
  [F_f_ref] -> To Workspace10/1
  [F_r_ref] -> To Workspace11/1
  [F_Tf] -> To Workspace12/1
  [F_Tf_ref] -> To Workspace13/1
  [F_Tr] -> To Workspace14/1
  [F_Tr_ref] -> To Workspace15/1
  [F_brf] -> To Workspace16/1
  [F_brf_ref] -> To Workspace17/1
  [F_brr] -> To Workspace18/1
  [F_brr_ref] -> To Workspace19/1
  [T_EDf] -> To Workspace20/1
  [T_EDf_ref] -> To Workspace21/1
  [T_EDr] -> To Workspace22/1
  [T_EDr_ref] -> To Workspace23/1
  [W_EDf] -> To Workspace24/1
  [W_EDr] -> To Workspace25/1
  [i_EDf] -> To Workspace26/1
  [i_EDr] -> To Workspace27/1
  Clock/1 -> To Workspace28/1
  Constant/1 -> Sum1/2
  [T_cell] -> Sum1/1
  Sum1/1 -> To Workspace29/1
  [T_EDf_trac_max] -> To Workspace33/1
  [T_EDf_gen_max] -> To Workspace34/1
  [T_EDr_trac_max] -> To Workspace35/1
  [T_EDr_gen_max] -> To Workspace36/1
  [T_EDf_ref] -> Relational Operator1/1, Relational Operator/1
  [T_EDf_trac_max] -> Relational Operator/2
  [T_EDf_gen_max] -> Relational Operator1/2
  Relational Operator/1 -> Logical Operator/1
  Relational Operator1/1 -> Logical Operator/2
  Logical Operator/1 -> Data Type Conversion1/1
  Integrator/1 -> To Workspace37/1
  Integrator1/1 -> To Workspace38/1
  Logical Operator1/1 -> Data Type Conversion/1
  Relational Operator3/1 -> Logical Operator1/2
  Relational Operator2/1 -> Logical Operator1/1
  [T_EDr_gen_max] -> Relational Operator3/2
  [T_EDr_trac_max] -> Relational Operator2/2
  [T_EDr_ref] -> Relational Operator2/1, Relational Operator3/1
  Data Type Conversion/1 -> Integrator1/1
  Data Type Conversion1/1 -> Integrator/1
  [T_cell] -> Relational Operator5/1, Relational Operator4/1
  Constant2/1 -> Relational Operator4/2
  Constant3/1 -> Relational Operator5/2
  Data Type Conversion2/1 -> Integrator2/1
  Logical Operator2/1 -> Data Type Conversion2/1
  Integrator2/1 -> To Workspace39/1
  Relational Operator4/1 -> Logical Operator2/1
  Relational Operator5/1 -> Logical Operator2/2

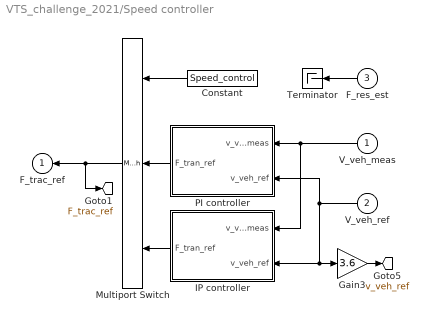
== system VTS_challenge_2021/Speed controller ==
  V_veh_meas : Inport
  V_veh_ref : Inport  Port=2
  F_res_est : Inport  Port=3
  Constant : Constant  Value=Speed_control
  Gain3 : Gain  Gain=3.6
  IP controller : Subsystem
  Multiport Switch : MultiPortSwitch  Inputs=2
  PI controller : Subsystem
  Terminator : Terminator
  F_trac_ref : Outport  InitialOutput=0
  tag scope: F_trac_ref=global, v_veh_ref=global
  wires:
  Multiport Switch/1 -> [F_trac_ref], F_trac_ref/1
  F_res_est/1 -> Terminator/1
  IP controller/1(F_tran_ref) -> Multiport Switch/3
  Constant/1 -> Multiport Switch/1
  V_veh_meas/1 -> IP controller/1(v_veh_meas), PI controller/1(v_veh_meas)
  PI controller/1(F_tran_ref) -> Multiport Switch/2
  Gain3/1 -> [v_veh_ref]
  V_veh_ref/1 -> Gain3/1, IP controller/2(v_veh_ref), PI controller/2(v_veh_ref)

== system VTS_challenge_2021/Battery/Air ==
  q_sa : Inport
  Constant : Constant  Value=BAT.T_air
  Terminator : Terminator
  T_air : Outport  InitialOutput=0
  wires:
  Constant/1 -> T_air/1
  q_sa/1 -> Terminator/1

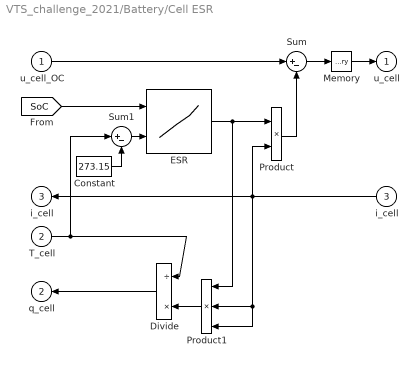
== system VTS_challenge_2021/Battery/Cell ESR ==
  u_cell_OC : Inport
  T_cell : Inport  Port=2
  "i_cell " : Inport  Port=3
  Constant : Constant  Value=273.15
  Divide : Product  Inputs=/*
  "ESR   " : Lookup_n-D  BreakpointsForDimension1=BAT.r_cell_SoC  BreakpointsForDimension2=BAT.r_cell_Temp  Table=BAT.r_cell  InternalRulePriority=Speed  RndMeth=Simplest  InputSameDT=on
  Memory : Memory  InitialCondition=BAT.v_cell_nom
  Product : Product
  Product1 : Product  Inputs=3
  Sum : Sum  Inputs=|+-
  Sum1 : Sum  Inputs=|+-
  u_cell : Outport  InitialOutput=0
  q_cell : Outport  Port=2  InitialOutput=0
  i_cell : Outport  Port=3  InitialOutput=0
  wires:
  [SoC] -> "ESR   "/1
  "ESR   "/1 -> Product1/1, Product/1
  "i_cell "/1 -> Product/2, Product1/2, Product1/3, i_cell/1
  u_cell_OC/1 -> Sum/1
  Product/1 -> Sum/2
  Sum/1 -> Memory/1
  Divide/1 -> q_cell/1
  Product1/1 -> Divide/2
  Memory/1 -> u_cell/1
  Constant/1 -> Sum1/2
  T_cell/1 -> Sum1/1, Divide/1
  Sum1/1 -> "ESR   "/2

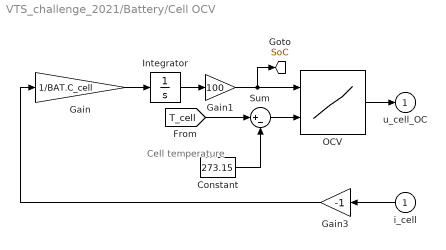
== system VTS_challenge_2021/Battery/Cell OCV ==
  note: Cell temperature
  i_cell : Inport
  Constant : Constant  Value=273.15
  Gain : Gain  Gain=1/BAT.C_cell
  Gain1 : Gain  Gain=100
  Gain3 : Gain  Gain=-1
  Integrator : Integrator  InitialCondition=BAT.SoC_init/100
  "OCV   " : Lookup_n-D  BreakpointsForDimension1=BAT.SoC  BreakpointsForDimension2=BAT.r_cell_Temp  Table=BAT.OCV  InternalRulePriority=Speed  RndMeth=Simplest  InputSameDT=on
  Sum : Sum  Inputs=|+-
  u_cell_OC : Outport  InitialOutput=0
  tag scope: SoC=global
  wires:
  i_cell/1 -> Gain3/1
  "OCV   "/1 -> u_cell_OC/1
  Gain/1 -> Integrator/1
  Gain3/1 -> Gain/1
  Gain1/1 -> "OCV   "/1, [SoC]
  Integrator/1 -> Gain1/1
  [T_cell] -> Sum/1
  Sum/1 -> "OCV   "/2
  Constant/1 -> Sum/2

== system VTS_challenge_2021/Battery/Series parallel connection ==
  u_cell : Inport
  i_bat : Inport  Port=2
  Gain2 : Gain  Gain=1/BAT.n_pa
  Gain4 : Gain  Gain=BAT.n_se
  u_bat : Outport  InitialOutput=0
  "i_cell " : Outport  Port=2  InitialOutput=0
  wires:
  Gain2/1 -> "i_cell "/1
  i_bat/1 -> Gain2/1
  Gain4/1 -> u_bat/1
  u_cell/1 -> Gain4/1

== system VTS_challenge_2021/Battery/Thermal capacitance ==
  q_cell : Inport
  q_cs : Inport  Port=2
  Constant : Constant  Value=BAT.Temp_0
  Divide : Product  Inputs=**
  Gain : Gain  Gain=1/BAT.C_th
  Integrator : Integrator
  Math Function : Math  SignedPower=on  SaturateOnIntegerOverflow=on
  Subtract : Sum  Inputs=+-
  T_cell : Outport  InitialOutput=0
  " T_cell " : Outport  Port=2  InitialOutput=0
  tag scope: T_cell=global
  wires:
  q_cell/1 -> Subtract/1
  q_cs/1 -> Subtract/2
  Subtract/1 -> Gain/1
  Gain/1 -> Integrator/1
  Constant/1 -> Divide/2
  Integrator/1 -> Math Function/1
  Math Function/1 -> Divide/1
  Divide/1 -> [T_cell], " T_cell "/1, T_cell/1

== system VTS_challenge_2021/Battery/Thermal resistance ==
  T_cell : Inport
  T_air : Inport  Port=2
  Divide : Product  Inputs=*/
  Divide1 : Product  Inputs=*/
  Gain : Gain  Gain=BAT.r_th
  Gain1 : Gain  Gain=BAT.r_th
  Sum : Sum  Inputs=|+-
  q_sa : Outport  InitialOutput=0
  q_cs : Outport  Port=2  InitialOutput=0
  wires:
  T_cell/1 -> Gain/1, Sum/1
  T_air/1 -> Gain1/1, Sum/2
  Sum/1 -> Divide1/1, Divide/1
  Divide/1 -> q_cs/1
  Gain/1 -> Divide/2
  Gain1/1 -> Divide1/2
  Divide1/1 -> q_sa/1

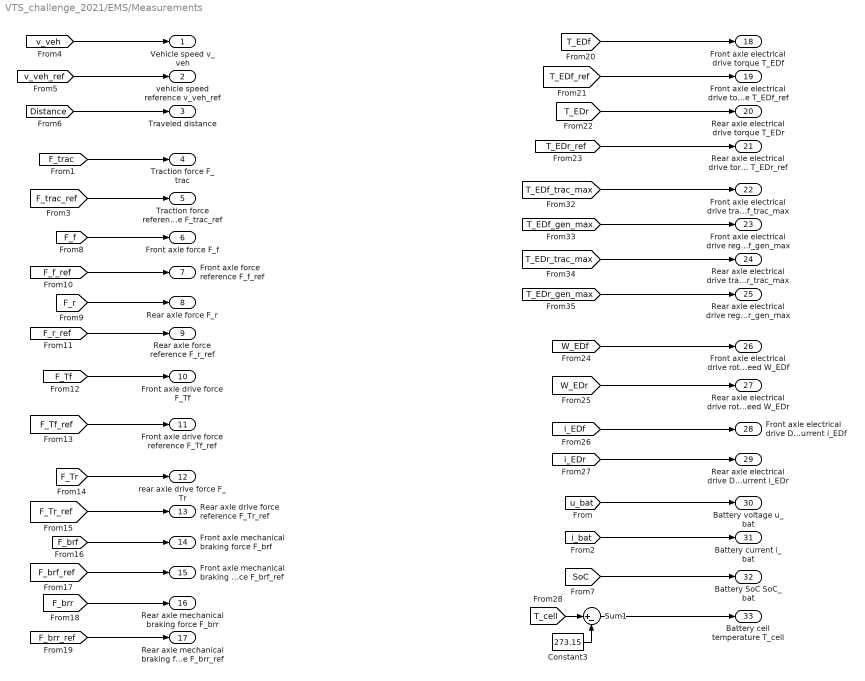
== system VTS_challenge_2021/EMS/Measurements ==
  Constant3 : Constant  Value=273.15
  Sum1 : Sum  Inputs=|+-
  Vehicle speed v_veh : Outport
  vehicle speed reference v_veh_ref : Outport  Port=2
  Traveled distance : Outport  Port=3
  Traction force F_trac : Outport  Port=4
  Traction force reference F_trac_ref : Outport  Port=5
  Front axle force F_f : Outport  Port=6
  Front axle force reference F_f_ref : Outport  Port=7
  Rear axle force F_r : Outport  Port=8
  Rear axle force reference F_r_ref : Outport  Port=9
  Front axle drive force F_Tf : Outport  Port=10
  Front axle drive force reference F_Tf_ref : Outport  Port=11
  rear axle drive force F_Tr : Outport  Port=12
  Rear axle drive force reference F_Tr_ref : Outport  Port=13
  Front axle mechanical braking force F_brf : Outport  Port=14
  Front axle mechanical braking force reference F_brf_ref : Outport  Port=15
  Rear axle mechanical braking force F_brr : Outport  Port=16
  Rear axle mechanical braking force reference F_brr_ref : Outport  Port=17
  Front axle electrical drive torque T_EDf : Outport  Port=18
  Front axle electrical drive torque reference T_EDf_ref : Outport  Port=19
  Rear axle electrical drive torque T_EDr : Outport  Port=20
  Rear axle electrical drive torque reference T_EDr_ref : Outport  Port=21
  Front axle electrical drive traction torque limitation T_EDf_trac_max : Outport  Port=22
  Front axle electrical drive regenerative torque limitation T_EDf_gen_max : Outport  Port=23
  Rear axle electrical drive traction torque limitation T_EDr_trac_max : Outport  Port=24
  Rear axle electrical drive regenerative torque limitation T_EDr_gen_max : Outport  Port=25
  Front axle electrical drive rotational speed W_EDf : Outport  Port=26
  Rear axle electrical drive rotational speed W_EDr : Outport  Port=27
  Front axle electrical drive DC bus current i_EDf : Outport  Port=28
  Rear axle electrical drive DC bus current i_EDr : Outport  Port=29
  Battery voltage u_bat : Outport  Port=30
  Battery current i_bat : Outport  Port=31
  Battery SoC SoC_bat : Outport  Port=32
  Battery cell temperature T_cell : Outport  Port=33
  wires:
  [F_trac_ref] -> Traction force reference F_trac_ref/1
  [F_brr] -> Rear axle mechanical braking force F_brr/1
  Constant3/1 -> Sum1/2
  [T_EDr_gen_max] -> Rear axle electrical drive regenerative torque limitation T_EDr_gen_max/1
  [W_EDr] -> Rear axle electrical drive rotational speed W_EDr/1
  [F_brf_ref] -> Front axle mechanical braking force reference F_brf_ref/1
  [v_veh_ref] -> vehicle speed reference v_veh_ref/1
  [T_EDr_trac_max] -> Rear axle electrical drive traction torque limitation T_EDr_trac_max/1
  [T_cell] -> Sum1/1
  [T_EDf_ref] -> Front axle electrical drive torque reference T_EDf_ref/1
  [F_brr_ref] -> Rear axle mechanical braking force reference F_brr_ref/1
  [F_r] -> Rear axle force F_r/1
  [F_r_ref] -> Rear axle force reference F_r_ref/1
  [Distance] -> Traveled distance/1
  [W_EDf] -> Front axle electrical drive rotational speed W_EDf/1
  [v_veh] -> Vehicle speed v_veh/1
  [i_EDf] -> Front axle electrical drive DC bus current i_EDf/1
  [F_Tr] -> rear axle drive force F_Tr/1
  [F_f] -> Front axle force F_f/1
  [F_Tf] -> Front axle drive force F_Tf/1
  [T_EDr] -> Rear axle electrical drive torque T_EDr/1
  [T_EDf_gen_max] -> Front axle electrical drive regenerative torque limitation T_EDf_gen_max/1
  [T_EDf_trac_max] -> Front axle electrical drive traction torque limitation T_EDf_trac_max/1
  Sum1/1 -> Battery cell temperature T_cell/1
  [SoC] -> Battery SoC SoC_bat/1
  [F_Tr_ref] -> Rear axle drive force reference F_Tr_ref/1
  [u_bat] -> Battery voltage u_bat/1
  [F_brf] -> Front axle mechanical braking force F_brf/1
  [T_EDr_ref] -> Rear axle electrical drive torque reference T_EDr_ref/1
  [i_EDr] -> Rear axle electrical drive DC bus current i_EDr/1
  [F_trac] -> Traction force F_trac/1
  [F_f_ref] -> Front axle force reference F_f_ref/1
  [F_Tf_ref] -> Front axle drive force reference F_Tf_ref/1
  [i_bat] -> Battery current i_bat/1
  [T_EDf] -> Front axle electrical drive torque T_EDf/1

== system VTS_challenge_2021/Speed controller/IP controller ==
  v_veh_meas : Inport
  v_veh_ref : Inport  Port=2
  Gain : Gain  Gain=SPEEDCONTROL.Kp_ip
  Gain1 : Gain  Gain=SPEEDCONTROL.Ki_ip
  Integrator : Integrator
  Sum1 : Sum  Inputs=-+
  Sum3 : Sum  Inputs=+-
  F_tran_ref : Outport
  wires:
  v_veh_ref/1 -> Sum1/2
  Gain/1 -> Sum3/2
  Integrator/1 -> Gain1/1
  v_veh_meas/1 -> Sum1/1, Gain/1
  Gain1/1 -> Sum3/1
  Sum3/1 -> F_tran_ref/1
  Sum1/1 -> Integrator/1

== system VTS_challenge_2021/Speed controller/PI controller ==
  v_veh_meas : Inport
  v_veh_ref : Inport  Port=2
  Gain : Gain  Gain=SPEEDCONTROL.Kp_pi
  Gain1 : Gain  Gain=SPEEDCONTROL.Ki_pi
  Integrator : Integrator
  Sum1 : Sum  Inputs=-+
  Sum3 : Sum
  F_tran_ref : Outport
  wires:
  Sum1/1 -> Gain/1, Integrator/1
  Sum3/1 -> F_tran_ref/1
  Gain1/1 -> Sum3/1
  v_veh_meas/1 -> Sum1/1
  Integrator/1 -> Gain1/1
  Gain/1 -> Sum3/2
  v_veh_ref/1 -> Sum1/2
